simulink model "gtm_design"  (R2021b)
settings: Solver=VariableStepAuto  StartTime=0.0  StopTime=30  MinStep=0.0049  RelTol=1e-3
StopFcn:
  | MWSout=grabmws(bdroot);
  | MWSout.lastrun=datestr(now);
values from neighbouring files (symbols this model uses):
  g = 32.17405    [SingleDOF.m]    (also in layer1atm.m; mainSimple.m = 32.174; simio.m = [dx(Index.EOM(1:6)); delta(:)-f; -delta(:)-f ])
  GuidanceMode = 1    [mainSimple.m]    (also in setup.m)
  knots2fps = 1/fps2knots    (= 1.687800745)    [main.m]    (also in mainSimple.m = 1.68781)
  s = tf('s')    [SingleDOF.m]    (also in main.m; mainSimple.m; newmain.m)
undefined symbols (not defined in the file or in its folder): Aero, aftfuel, aftfuel_pos, AILL, AILLC, AILR, AILRC, alpha_deg, altitude_ft, Ax_g, Ay_g, Az_g, b, beta_deg, bias, BRAKEC, Cbar, cg_pos0, cg_shift_gear, DamageCase, DamageModels, DamageOnsetTime, Earth, ELLIB, ELLIBC, ELLOB, ELLOBC, ELRIB, ELRIBC, ELROB, ELROBC, engl_ang, engl_pos, engr_ang, engr_pos, FLAPLC, FLAPLIB, FLAPLOB, FLAPRC, FLAPRIB, FLAPROB, FuelUsed_Init, fwdfuel, fwdfuel_pos, GEAR, GEARC, Inertia0, Inertia_shift_gear, Ixx_model, Iyy_model, Izz_model, KTAS, LandingGear, LengON, LinearizeModeOn, m, MORPHLC, MORPHRC, NAV_altitude_m, NAV_latitude_deg ... (+51)
libraries: simulink_extras x39, simulink_need_slupdate x30, LPVBlockLibrary x9, aerolibconvert2 x7, simulink x3, aerolibtransform2 x3, UserContent_lib x2, uavalgslib x2, robotcorelib x1, uavutilslib x1
(part 7 of 7)

== system gtm_design/GTM_T2/Aero/Dynamic Derviatives/Rotary Blended UnDamaged Case/Forced Oscillation ==
  alpha : Inport
  pqr : Inport  Port=2
  Assignment to Lateral : Assignment  IndexMode=Zero-based  IndexOptions=Index vector (dialog)  Indices=[1 3 5]  OutputSizes=[1 1]
  Assignment to Lateral1 : Assignment  IndexMode=Zero-based  IndexOptions=Index vector (dialog)  Indices=[1 3 5]  OutputSizes=[1 1]
  Assignment to Longitudinal : Assignment  IndexMode=Zero-based  IndexOptions=Index vector (dialog)  Indices=[0 2 4]  OutputSizes=[1 1]
  Constant : Constant  Value=zeros(6,1)
  Constant1 : Constant  Value=[0:2]  OutDataTypeStr=uint32
  Constant2 : Constant  Value=[0:2]  OutDataTypeStr=uint32
  Constant3 : Constant  Value=[0:2]  OutDataTypeStr=uint32
  Constant4 : Constant  Value=zeros(6,1)
  Constant5 : Constant  Value=zeros(6,1)
  Demux : Demux  Outputs=3
  PreLookup Index Search : simulink_need_slupdate/PreLookup Index Search  bpData=Aero.dC3_q.alpha  searchMode=Binary Search  cacheBpFlag=on  outputFlag=off  IndexDataType=uint32  extrapMode=Linear Extrapolation  rangeErrorMode=None
      settings: SourceProductBaseCode=SL
  PreLookup Index Search1 : simulink_need_slupdate/PreLookup Index Search  bpData=Aero.dC3_r.rhat  searchMode=Binary Search  cacheBpFlag=on  outputFlag=off  IndexDataType=uint32  extrapMode=Linear Extrapolation  rangeErrorMode=None
      settings: SourceProductBaseCode=SL
  PreLookup Index Search2 : simulink_need_slupdate/PreLookup Index Search  bpData=Aero.dC3_p.phat  searchMode=Binary Search  cacheBpFlag=on  outputFlag=off  IndexDataType=uint32  extrapMode=Linear Extrapolation  rangeErrorMode=None
      settings: SourceProductBaseCode=SL
  PreLookup Index Search3 : simulink_need_slupdate/PreLookup Index Search  bpData=Aero.dC3_q.qhat  searchMode=Binary Search  cacheBpFlag=on  outputFlag=off  IndexDataType=uint32  extrapMode=Linear Extrapolation  rangeErrorMode=None
      settings: SourceProductBaseCode=SL
  PreLookup Index Search4 : simulink_need_slupdate/PreLookup Index Search  bpData=Aero.dC3_p.alpha  searchMode=Binary Search  cacheBpFlag=on  outputFlag=off  IndexDataType=uint32  extrapMode=Linear Extrapolation  rangeErrorMode=None
      settings: SourceProductBaseCode=SL
  PreLookup Index Search5 : simulink_need_slupdate/PreLookup Index Search  bpData=Aero.dC3_r.alpha  searchMode=Binary Search  cacheBpFlag=on  outputFlag=off  IndexDataType=uint32  extrapMode=Linear Extrapolation  rangeErrorMode=None
      settings: SourceProductBaseCode=SL
  pitch : simulink_need_slupdate/Interpolation (n-D) using PreLookup  numDimsPopupSelect=3  explicitNumDims=2  table=Aero.dC3_q.data  interpMethod=Linear  extrapMethod=Linear  rangeErrorMode=None  NumSelectionDims=1
      settings: SourceProductBaseCode=SL
  roll : simulink_need_slupdate/Interpolation (n-D) using PreLookup  numDimsPopupSelect=3  explicitNumDims=2  table=Aero.dC3_p.data  interpMethod=Linear  extrapMethod=Linear  rangeErrorMode=None  NumSelectionDims=1
      settings: SourceProductBaseCode=SL
  yaw : simulink_need_slupdate/Interpolation (n-D) using PreLookup  numDimsPopupSelect=3  explicitNumDims=2  table=Aero.dC3_r.data  interpMethod=Linear  extrapMethod=Linear  rangeErrorMode=None  NumSelectionDims=1
      settings: SourceProductBaseCode=SL
  dC6_p : Outport
  dC6_q : Outport  Port=2
  dC6_r : Outport  Port=3
  wires:
  alpha/1 -> PreLookup Index Search4/1, PreLookup Index Search5/1, PreLookup Index Search/1
  pqr/1 -> Demux/1
  Constant1/1 -> pitch/3
  Demux/2 -> PreLookup Index Search3/1
  Demux/1 -> PreLookup Index Search2/1
  Demux/3 -> PreLookup Index Search1/1
  Constant2/1 -> roll/3
  Constant3/1 -> yaw/3
  Constant/1 -> Assignment to Longitudinal/1
  pitch/1 -> Assignment to Longitudinal/2
  roll/1 -> Assignment to Lateral/2
  Constant4/1 -> Assignment to Lateral/1
  Constant5/1 -> Assignment to Lateral1/1
  yaw/1 -> Assignment to Lateral1/2
  PreLookup Index Search1/1 -> yaw/2
  PreLookup Index Search2/1 -> roll/2
  PreLookup Index Search3/1 -> pitch/2
  Assignment to Lateral/1 -> dC6_p/1
  Assignment to Lateral1/1 -> dC6_r/1
  Assignment to Longitudinal/1 -> dC6_q/1
  PreLookup Index Search/1 -> pitch/1
  PreLookup Index Search4/1 -> roll/1
  PreLookup Index Search5/1 -> yaw/1

== system gtm_design/GTM_T2/Aero/Dynamic Derviatives/Rotary Blended UnDamaged Case/Rotary Balance ==
  alpha : Inport
  beta : Inport  Port=2
  w : Inport  Port=3
  Constant1 : Constant  Value=[0:5]  OutDataTypeStr=uint32
  PreLookup Index Search : simulink_need_slupdate/PreLookup Index Search  bpData=Aero.dC6_w.alpha  searchMode=Binary Search  cacheBpFlag=on  outputFlag=off  IndexDataType=uint32  extrapMode=Linear Extrapolation  rangeErrorMode=None
      settings: SourceProductBaseCode=SL
  PreLookup Index Search1 : simulink_need_slupdate/PreLookup Index Search  bpData=Aero.dC6_w.beta  searchMode=Binary Search  cacheBpFlag=on  outputFlag=off  IndexDataType=uint32  extrapMode=Linear Extrapolation  rangeErrorMode=None
      settings: SourceProductBaseCode=SL
  PreLookup Index Search2 : simulink_need_slupdate/PreLookup Index Search  bpData=Aero.dC6_w.what  searchMode=Binary Search  cacheBpFlag=on  outputFlag=off  IndexDataType=uint32  extrapMode=Linear Extrapolation  rangeErrorMode=None
      settings: SourceProductBaseCode=SL
  TableLookup : simulink_need_slupdate/Interpolation (n-D) using PreLookup  numDimsPopupSelect=4  explicitNumDims=2  table=Aero.dC6_w.data  interpMethod=Linear  extrapMethod=Linear  rangeErrorMode=None  NumSelectionDims=1
      settings: SourceProductBaseCode=SL
  dC6 : Outport
  wires:
  PreLookup Index Search/1 -> TableLookup/1
  beta/1 -> PreLookup Index Search1/1
  alpha/1 -> PreLookup Index Search/1
  TableLookup/1 -> dC6/1
  Constant1/1 -> TableLookup/4
  w/1 -> PreLookup Index Search2/1
  PreLookup Index Search1/1 -> TableLookup/3
  PreLookup Index Search2/1 -> TableLookup/2

== system gtm_design/GTM_T2/Sensors/Air Data/First Order Filter/Enabled Subsystem ==
  In : Inport
  tau : Inport  Port=2
  Enable : EnablePort
  Divide : Product  Inputs=*/
  Integrator : Integrator  InitialConditionSource=external  UpperSaturationLimit=POS_hi  LowerSaturationLimit=POS_lo
  Sum : Sum  Inputs=-+|  InputSameDT=on  SaturateOnIntegerOverflow=on  OutDataTypeStr=Inherit: Same as first input
  Out : Outport
  wires:
  Sum/1 -> Divide/1  "Error"
  In/1 -> Sum/2, Integrator/2
  Integrator/1 -> Out/1, Sum/1  "Y"
  tau/1 -> Divide/2
  Divide/1 -> Integrator/1  "Ydot"

== system gtm_design/GTM_T2/TransportDelay/Transport Delay on Bus/BusDelay/TimeDelay with IC feedthrough ==
  I : Inport
  Clock : Clock
  Switch : Switch  Criteria=u2 > Threshold  Threshold=TimeDelay
  Transport Delay : TransportDelay  DelayTime=TimeDelay
      settings: AttributesFormatString=%<DelayTime>
  O : Outport
  wires:
  I/1 -> Transport Delay/1, Switch/3
  Clock/1 -> Switch/2
  Switch/1 -> O/1
  Transport Delay/1 -> Switch/1

== system gtm_design/GTM_T2/TransportDelay/Transport Delay on Bus/BusDelay1/TimeDelay with IC feedthrough ==
  I : Inport
  Clock : Clock
  Switch : Switch  Criteria=u2 > Threshold  Threshold=TimeDelay
  Transport Delay : TransportDelay  DelayTime=TimeDelay
      settings: AttributesFormatString=%<DelayTime>
  O : Outport
  wires:
  I/1 -> Transport Delay/1, Switch/3
  Clock/1 -> Switch/2
  Switch/1 -> O/1
  Transport Delay/1 -> Switch/1

== system gtm_design/GTM_T2/TransportDelay/Transport Delay on Bus/BusDelay2/TimeDelay with IC feedthrough ==
  I : Inport
  Clock : Clock
  Switch : Switch  Criteria=u2 > Threshold  Threshold=TimeDelay
  Transport Delay : TransportDelay  DelayTime=TimeDelay
      settings: AttributesFormatString=%<DelayTime>
  O : Outport
  wires:
  I/1 -> Transport Delay/1, Switch/3
  Clock/1 -> Switch/2
  Switch/1 -> O/1
  Transport Delay/1 -> Switch/1

== system gtm_design/GTM_T2/TransportDelay/Transport Delay on Bus/BusDelay3/TimeDelay with IC feedthrough ==
  I : Inport
  Clock : Clock
  Switch : Switch  Criteria=u2 > Threshold  Threshold=TimeDelay
  Transport Delay : TransportDelay  DelayTime=TimeDelay
      settings: AttributesFormatString=%<DelayTime>
  O : Outport
  wires:
  I/1 -> Transport Delay/1, Switch/3
  Clock/1 -> Switch/2
  Switch/1 -> O/1
  Transport Delay/1 -> Switch/1

== system gtm_design/GTM_T2/TransportDelay/Transport Delay on Bus/BusDelay4/TimeDelay with IC feedthrough ==
  I : Inport
  Clock : Clock
  Switch : Switch  Criteria=u2 > Threshold  Threshold=TimeDelay
  Transport Delay : TransportDelay  DelayTime=TimeDelay
      settings: AttributesFormatString=%<DelayTime>
  O : Outport
  wires:
  I/1 -> Transport Delay/1, Switch/3
  Clock/1 -> Switch/2
  Switch/1 -> O/1
  Transport Delay/1 -> Switch/1

== system gtm_design/Control/Controller/Control Algorithm/Longitudinal Controller/Altitude Controller/Altitude Controller ==
  alt_c_ft : Inport
  feedback : Inport  Port=2
  An_c_g : Step  Time=5  Before=0.9968  After=0.9  SampleTime=0
  An_c_g1 : Step  Time=10  After=0.0968  SampleTime=0
  Constant : Constant  Commented=on
  Constant1 : Constant  Value=0.9968
  Gain : Gain  Gain=-1
  Sum : Sum  Inputs=|++
  Terminator : Terminator
  Terminator1 : Terminator
  Az_c_g : Outport
  wires:
  alt_c_ft/1 -> Terminator/1
  feedback/1 -> Terminator1/1
  Gain/1 -> Az_c_g/1  "Az_c_g"
  An_c_g/1 -> Sum/1
  An_c_g1/1 -> Sum/2
  Sum/1 -> Gain/1

== system gtm_design/Control/Controller/Control Algorithm/Longitudinal Controller/Altitude Controller/Normal Acceleration Controller ==
  Az_c_g : Inport
  feedback : Inport  Port=2
  Demux2 : Demux  Outputs=[2 1]
  Full Output : Subsystem
  LPV Controller : LPVBlockLibrary/LPVBlock  sys=K_lon_lpv  plist={'rho1_sas_param';'rho2_alt_param';'rho3_mor_param'}  x0=0
      settings: SourceProductName=LPVTools Blocks
  Mux : Mux  Inputs=2
  Scheduling Parameter : Subsystem
  Scope : Scope
  Scope1 : Scope
  Scope2 : Scope
  Sum : Sum  Inputs=|+-
  Sum1 : Sum  Inputs=|+-
  Sum2 : Sum  Inputs=|++
  Sum3 : Sum  Inputs=|+-
  Trim Command : Subsystem
  Trim Input : Subsystem
  Trim Output : Subsystem
  dele_c_deg : Scope
  feedback_1 : InportShadow  Port=2
  knotstofps : Gain  Gain=g
  ELLC : Outport
  wires:
  feedback/1 -> Scheduling Parameter/1(feedback)
  Mux/1 -> LPV Controller/1
  [rho] -> Trim Input/1(rho)
  LPV Controller/1 -> Sum2/1  "du"
  Scheduling Parameter/1(rho) -> [rho]
  Sum3/1 -> Scope2/1, Mux/1  "dy"
  Sum1/1 -> Demux2/1  "dx"
  Trim Input/1(dele_trim_deg) -> Sum2/2
  Sum2/1 -> ELLC/1, dele_c_deg/1  "u"
  feedback_1/1 -> Full Output/1(feedback)
  [rho] -> Trim Output/1(rho)
  Trim Output/1(y_eq) -> Sum1/2  "y_eq"
  [rho] -> LPV Controller/2
  Full Output/1(y) -> Sum1/1  "y"
  Az_c_g/1 -> knotstofps/1
  knotstofps/1 -> Sum/1  "Az_c_fps"
  Trim Command/1(Az_trim_fps) -> Sum/2
  Sum/1 -> Scope/1, Sum3/1
  Demux2/2 -> Sum3/2, Scope1/1
  Demux2/1 -> Mux/2

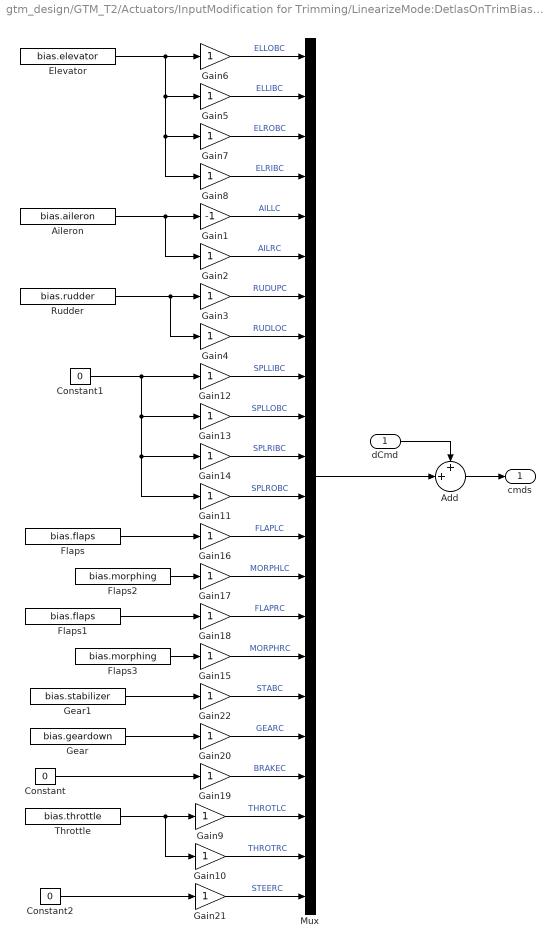
== system gtm_design/GTM_T2/Actuators/InputModification for Trimming/LinearizeMode:DetlasOnTrimBias/Surface Allocation For Linearizing/BiasSurfs ==
  dCmd : Inport
  Add : Sum  Inputs=++|
  Aileron : Constant  Value=bias.aileron
  Constant : Constant  Value=0
  Constant1 : Constant  Value=0
  Constant2 : Constant  Value=0
  Elevator : Constant  Value=bias.elevator
  Flaps : Constant  Value=bias.flaps
  Flaps1 : Constant  Value=bias.flaps
  Flaps2 : Constant  Value=bias.morphing
  Flaps3 : Constant  Value=bias.morphing
  Gain1 : Gain  Gain=-1  SaturateOnIntegerOverflow=on  OutDataTypeStr=Inherit: Same as input  ParamDataTypeStr=Inherit: Same as input
  Gain{2..22} (21 alike) : Gain  SaturateOnIntegerOverflow=on  OutDataTypeStr=Inherit: Same as input  ParamDataTypeStr=Inherit: Same as input
  Gear : Constant  Value=bias.geardown
  Gear1 : Constant  Value=bias.stabilizer
  Mux : Mux  Inputs=22
  Rudder : Constant  Value=bias.rudder
  Throttle : Constant  Value=bias.throttle
  cmds : Outport
  wires:
  Gain21/1 -> Mux/22  "STEERC"
  Constant2/1 -> Gain21/1
  Throttle/1 -> Gain10/1, Gain9/1
  Gain10/1 -> Mux/21  "THROTRC"
  Gain9/1 -> Mux/20  "THROTLC"
  Add/1 -> cmds/1
  dCmd/1 -> Add/1
  Mux/1 -> Add/2
  Gain22/1 -> Mux/17  "STABC"
  Gear1/1 -> Gain22/1
  Aileron/1 -> Gain2/1, Gain1/1
  Gain2/1 -> Mux/6  "AILRC"
  Gain1/1 -> Mux/5  "AILLC"
  Gain20/1 -> Mux/18  "GEARC"
  Constant/1 -> Gain19/1
  Gear/1 -> Gain20/1
  Gain19/1 -> Mux/19  "BRAKEC"
  Flaps/1 -> Gain16/1
  Rudder/1 -> Gain4/1, Gain3/1
  Elevator/1 -> Gain8/1, Gain7/1, Gain5/1, Gain6/1
  Gain4/1 -> Mux/8  "RUDLOC"
  Gain3/1 -> Mux/7  "RUDUPC"
  Gain8/1 -> Mux/4  "ELRIBC"
  Gain7/1 -> Mux/3  "ELROBC"
  Gain6/1 -> Mux/1  "ELLOBC"
  Gain5/1 -> Mux/2  "ELLIBC"
  Gain15/1 -> Mux/16  "MORPHRC"
  Gain18/1 -> Mux/15  "FLAPRC"
  Gain17/1 -> Mux/14  "MORPHLC"
  Gain16/1 -> Mux/13  "FLAPLC"
  Gain11/1 -> Mux/12  "SPLROBC"
  Gain14/1 -> Mux/11  "SPLRIBC"
  Gain13/1 -> Mux/10  "SPLLOBC"
  Gain12/1 -> Mux/9  "SPLLIBC"
  Constant1/1 -> Gain13/1, Gain11/1, Gain14/1, Gain12/1
  Flaps2/1 -> Gain17/1
  Flaps1/1 -> Gain18/1
  Flaps3/1 -> Gain15/1

== system gtm_design/GTM_T2/Actuators/InputModification for Trimming/TrimMode: DriveFromTopLevel/MapPitchSurf/UseElevatorToTrim ==
  In : Inport
  Action Port : ActionPort  ActionPortLabel=default:
  Constant1 : Constant  Value=bias.stabilizer
  Gain : Gain  Gain=[1;1;1;1]
  Mux : Mux  Inputs=[4 1]
  Out : Outport  InitialOutput=[0;0;0;0;bias.stabilizer]
  wires:
  Mux/1 -> Out/1
  Gain/1 -> Mux/1
  Constant1/1 -> Mux/2
  In/1 -> Gain/1

== system gtm_design/GTM_T2/Actuators/InputModification for Trimming/TrimMode: DriveFromTopLevel/MapPitchSurf/UseStabToTrim ==
  In : Inport
  Action Port : ActionPort  ActionPortLabel=case [ 1 ]:
  Constant1 : Constant  Value=bias.elevator
  Gain2 : Gain  Gain=[1;1;1;1]
  Mux : Mux  Inputs=[4 1]
  Out1 : Outport  InitialOutput=[bias.elevator*[1;1;1;1];0]
  wires:
  Mux/1 -> Out1/1
  Gain2/1 -> Mux/1
  In/1 -> Mux/2
  Constant1/1 -> Gain2/1

== system gtm_design/Control/Controller/Control Algorithm/Longitudinal Controller/Altitude Controller/Normal Acceleration Controller/Full Output ==
  feedback : Inport
  Az_g : Scope
  Bus Selector : BusSelector  OutputSignals=AirData.alpha_deg,MAG3.q_deg,MAG3.Az_g
  Degrees to Radians : simulink_extras/Transformations/Degrees to Radians
  Degrees to Radians1 : simulink_extras/Transformations/Degrees to Radians
  Mux : Mux  Inputs=3
  alpha_deg : Scope
  knotstofps : Gain  Gain=g
  q_deg : Scope
  y : Outport
  wires:
  feedback/1 -> Bus Selector/1
  Bus Selector/1 -> alpha_deg/1, Degrees to Radians/1  "<alpha_deg>"
  Bus Selector/2 -> q_deg/1, Degrees to Radians1/1  "<q_deg>"
  Bus Selector/3 -> knotstofps/1, Az_g/1  "<Az_g>"
  Degrees to Radians1/1 -> Mux/2  "q_rad"
  Degrees to Radians/1 -> Mux/1  "alp_rad"
  knotstofps/1 -> Mux/3  "Az_fps"
  Mux/1 -> y/1

== system gtm_design/Control/Controller/Control Algorithm/Longitudinal Controller/Altitude Controller/Normal Acceleration Controller/Scheduling Parameter ==
  feedback : Inport
  Add : Sum
  Bus Selector1 : BusSelector  OutputSignals=AirData.KTAS,MIDG.NAV_altitude_m,SurfacePos.FLAPLOB,SurfacePos.FLAPROB  OutputAsBus=on
  Bus to Vector : BusToVector
  Demux : Demux
  Gain : Gain  Gain=0.5
  Length Conversion : aerolibconvert2/Length Conversion  IU=m  OU=ft
  MATLAB Function : MATLAB Function  TreatAsAtomicUnit=on
  Mux : Mux  Inputs=3
  rho : Outport
  wires:
  feedback/1 -> Bus Selector1/1
  Bus Selector1/1 -> Bus to Vector/1
  Demux/3 -> Add/1
  Demux/1 -> MATLAB Function/1(tas)
  Demux/4 -> Add/2
  MATLAB Function/1(sas) -> Mux/1  "sas"
  Add/1 -> Gain/1
  Gain/1 -> Mux/3  "mor"
  Demux/2 -> Length Conversion/1  "alt"
  Bus to Vector/1 -> Demux/1
  Mux/1 -> rho/1
  Length Conversion/1 -> MATLAB Function/2(h), Mux/2

== system gtm_design/Control/Controller/Control Algorithm/Longitudinal Controller/Altitude Controller/Normal Acceleration Controller/Trim Command ==
  Constant : Constant  Value=-1
  knotstofps : Gain  Gain=g
  Az_trim_fps : Outport
  wires:
  knotstofps/1 -> Az_trim_fps/1  "Az_c_fps"
  Constant/1 -> knotstofps/1

== system gtm_design/Control/Controller/Control Algorithm/Longitudinal Controller/Altitude Controller/Normal Acceleration Controller/Trim Input ==
  rho : Inport
  Constant3 : Constant
  Scope1 : Scope
  dele_trim : LPVBlockLibrary/LPVBlock  sys=sch_elevator_trim  plist={'rho1_sas_param';'rho2_alt_param';'rho3_mor_param'}  x0=0
      settings: SourceProductName=LPVTools Blocks
  dele_trim_deg : Outport
  wires:
  Constant3/1 -> dele_trim/1
  dele_trim/1 -> dele_trim_deg/1, Scope1/1  "dele_trim_deg"
  rho/1 -> dele_trim/2

== system gtm_design/Control/Controller/Control Algorithm/Longitudinal Controller/Altitude Controller/Normal Acceleration Controller/Trim Output ==
  rho : Inport
  Constant1 : Constant  Value=0
  Constant2 : Constant
  Constant3 : Constant  Value=-1
  Degrees to Radians : simulink_extras/Transformations/Degrees to Radians
  LPVBlock : LPVBlockLibrary/LPVBlock  sys=sch_alp_trim  plist={'rho1_sas_param';'rho2_alt_param';'rho3_mor_param'}  x0=0
      settings: SourceProductName=LPVTools Blocks
  Mux : Mux  Inputs=3
  Scope : Scope
  knotstofps : Gain  Gain=g
  y_eq : Outport
  wires:
  Degrees to Radians/1 -> Mux/1  "alp_trim_rad"
  Constant2/1 -> LPVBlock/1
  LPVBlock/1 -> Scope/1, Degrees to Radians/1  "alp_trim_deg"
  Constant1/1 -> Mux/2  "q_trim_rad"
  knotstofps/1 -> Mux/3  "Az_trim_fps"
  rho/1 -> LPVBlock/2
  Constant3/1 -> knotstofps/1  "Az_trim_g"
  Mux/1 -> y_eq/1

== matlab function gtm_design/GTM_T2/EOM/Aircraft 6DOF/Form Inertia Matrix ==
  data: Ixx input double size=1; I output size=[3 3]; Iyy input size=1; Izz input size=1; Ixz input size=1; Iyz input size=1; Ixy input size=1; InvI output size=[3 3]
function [I,InvI] = Inertia(Ixx,Iyy,Izz,Ixz,Iyz,Ixy)
% This block supports an embeddable subset of the MATLAB language.
% See the help menu for details. 

I=[ Ixx, -Ixy, -Ixz;
   -Ixy,  Iyy, -Iyz;
   -Ixz, -Iyz,   Izz ];

det = Ixx*Iyy*Izz-Ixx*Iyz^2-Ixy^2*Izz-2*Ixy*Ixz*Iyz-Ixz^2*Iyy;

adjoint=[...
Iyy*Izz-Iyz^2,    Ixy*Izz+Ixz*Iyz, Ixy*Iyz+Ixz*Iyy;...
Ixy*Izz+Ixz*Iyz,   Ixx*Izz-Ixz^2,  Ixx*Iyz+Ixy*Ixz;...
Ixy*Iyz+Ixz*Iyy,  Ixx*Iyz+Ixy*Ixz,   Ixx*Iyy-Ixy^2     ];

InvI=adjoint/det;

== matlab function gtm_design/GTM_T2/Engines/Engine Alignment ==
  data: T output; Tl input; hl input; Tr input; hr input; TL output; engl_ang parameter; engr_ang parameter; TR output; H output
function [T,TL,TR,H] = eng_angles(Tl,hl,Tr,hr,engl_ang,engr_ang)
% This block supports an embeddable subset of the MATLAB language.
% See the help menu for details. 

% Using the engine alignment angles (set in AC_params_T2.m), compute the 
% off-axis thrust and angular momentum terms.

TL = Tl*[cosd(engl_ang(2))*cosd(engl_ang(3));...
         sind(engl_ang(3));...
         -sind(engl_ang(2))*cosd(engl_ang(3))];
TR = Tr*[cosd(engr_ang(2))*cosd(engr_ang(3));...
         sind(engr_ang(3));...
         -sind(engr_ang(2))*cosd(engr_ang(3))];  
T = TL+TR;

H = hl*[cosd(engl_ang(2))*cosd(engl_ang(3));...
         sind(engl_ang(3));...
         -sind(engl_ang(2))*cosd(engl_ang(3))] + ...
         hr*[cosd(engr_ang(2))*cosd(engr_ang(3));...
         sind(engr_ang(3));...
         -sind(engr_ang(2))*cosd(engr_ang(3))];

== matlab function gtm_design/GTM_T2/Engines/Left_Engine Jetcat P70/Simple Ram Drag Model ==
  data: ram_drag output; qbar input; S input; ram_drag_coef parameter
function ram_drag =   ram_drag(qbar,S,ram_drag_coef)
% This block supports the Embedded MATLAB subset.
% See the help menu for details. 

ram_drag = ram_drag_coef.*qbar.*S;
return

== matlab function gtm_design/GTM_T2/Engines/Right_Engine Jetcat P70/Simple Ram Drag Model ==
  data: ram_drag output; qbar input; S input; ram_drag_coef parameter
function ram_drag =   ram_drag(qbar,S,ram_drag_coef)
% This block supports the Embedded MATLAB subset.
% See the help menu for details. 

ram_drag = ram_drag_coef.*qbar.*S;
return

== matlab function gtm_design/Control/Controller/Control Algorithm/Longitudinal Controller (Gamma)/Scheduling Parameter/MATLAB Function ==
  data: tas input; sas output; h input
function sas = fcn(tas, h)
sas = 100-30000/(30000-h)*(100-tas);

== matlab function gtm_design/GTM_T2/A/C parameters/Inertia/Mass/CG Shift/FuelBurnEffects/Polyval1/Embedded MATLAB Function ==
  data: u input; y output; p parameter
function y = fcn(u,p)
% This block supports the Embedded MATLAB subset.
% See the help menu for details. 


y = sum(p.*u.^(length(p)-1:-1:0));

== matlab function gtm_design/Control/Controller/Control Algorithm/Longitudinal Controller (Gamma)/Trim Command/MATLAB Function ==
  data: sas input; tas output; h input
function tas = fcn(sas,h)

tas = 100-(30000-h)/30000*(100-sas);

== matlab function gtm_design/Control/Controller/Control Algorithm/Lateral-Directional Controller/Scheduling Parameter/MATLAB Function ==
  data: tas input; sas output; h input
function sas = fcn(tas, h)
sas = 100-30000/(30000-h)*(100-tas);

== matlab function gtm_design/GTM_T2/A//C parameters/Inertia//Mass//CG Shift/MorphingEffects/MorphingEffectsInertia ==
  data: fuel_used input; y output; aftfuel parameter; fwdfuel parameter; aftfuel_pos parameter; fwdfuel_pos parameter; w0 parameter; cg_pos0 parameter
function y = fcn(fuel_used,aftfuel,fwdfuel,aftfuel_pos,fwdfuel_pos,w0,cg_pos0)
% This block supports an embeddable subset of the MATLAB language.
% See the help menu for details. 

y = w0.*cg_pos0 - min(aftfuel,fuel_used).*aftfuel_pos - max(0,fuel_used-fwdfuel).*fwdfuel_pos;

== matlab function gtm_design/GTM_T2/A//C parameters/Inertia//Mass//CG Shift/MorphingEffects1/MorphingEffectsCG ==
  data: fuel_used input; y output; aftfuel parameter; fwdfuel parameter; aftfuel_pos parameter; fwdfuel_pos parameter; w0 parameter; cg_pos0 parameter
function y = fcn(fuel_used,aftfuel,fwdfuel,aftfuel_pos,fwdfuel_pos,w0,cg_pos0)
% This block supports an embeddable subset of the MATLAB language.
% See the help menu for details. 

y = w0.*cg_pos0 - min(aftfuel,fuel_used).*aftfuel_pos - max(0,fuel_used-fwdfuel).*fwdfuel_pos;

== matlab function gtm_design/Control/Controller/Control Algorithm/Longitudinal Controller (Gamma)/Trim State/MATLAB Function ==
  data: sas input; tas output; h input
function tas = fcn(sas,h)

tas = 100-(30000-h)/30000*(100-sas);

== matlab function gtm_design/Guidance/Orbit Following/Heading Control ==
  data: FlightState input Bus: FixedWingStateBus; UHeading input; RollAngle output size=[1 1]; e input Bus: FixedWingEnvironmentBus
function RollAngle = fcn(FlightState, UHeading, e)

PHeadingAngle = 0.39;

Va = FlightState.AirSpeed;
HeadingAngle = FlightState.HeadingAngle;
FlightPathAngle = FlightState.FlightPathAngle;

YawAngle = HeadingAngle - asin((1/Va)*[e.WindNorth, e.WindEast]*[-sin(HeadingAngle); cos(HeadingAngle)]);
b = [cos(HeadingAngle)*cos(FlightPathAngle), sin(HeadingAngle)*cos(FlightPathAngle), -sin(FlightPathAngle)]*[e.WindNorth; e.WindEast; e.WindDown];
c = [e.WindNorth, e.WindEast, e.WindDown]*[e.WindNorth; e.WindEast; e.WindDown]- Va^2;
Vg = -b+sqrt(b^2-c);

RollAngle = atan2(PHeadingAngle*angdiff(HeadingAngle,UHeading)*Vg,e.Gravity*cos(HeadingAngle-YawAngle));

== matlab function gtm_design/Guidance/Waypoint Following/Heading Control ==
  data: FlightState input Bus: FixedWingStateBus; UHeading input; RollAngle output size=[1 1]; e input Bus: FixedWingEnvironmentBus
function RollAngle = fcn(FlightState, UHeading, e)

PHeadingAngle = 0.39;

Va = FlightState.AirSpeed;
HeadingAngle = FlightState.HeadingAngle;
FlightPathAngle = FlightState.FlightPathAngle;

YawAngle = HeadingAngle - asin((1/Va)*[e.WindNorth, e.WindEast]*[-sin(HeadingAngle); cos(HeadingAngle)]);
b = [cos(HeadingAngle)*cos(FlightPathAngle), sin(HeadingAngle)*cos(FlightPathAngle), -sin(FlightPathAngle)]*[e.WindNorth; e.WindEast; e.WindDown];
c = [e.WindNorth, e.WindEast, e.WindDown]*[e.WindNorth; e.WindEast; e.WindDown]- Va^2;
Vg = -b+sqrt(b^2-c);

RollAngle = atan2(PHeadingAngle*angdiff(HeadingAngle,UHeading)*Vg,e.Gravity*cos(HeadingAngle-YawAngle));

== matlab function gtm_design/Control/Controller/Control Algorithm/Longitudinal Controller/Altitude Controller/Normal Acceleration Controller/Scheduling Parameter/MATLAB Function ==
  data: tas input; sas output; h input
function sas = fcn(tas, h)
sas = 100-30000/(30000-h)*(100-tas);

== matlab function gtm_design/GTM_T2/A/C parameters/Inertia/Mass/CG Shift/fuel cg shift, cg_pos0 ==
  data: fuel_used input; y output; aftfuel parameter; fwdfuel parameter; aftfuel_pos parameter; fwdfuel_pos parameter; w0 parameter; cg_pos0 parameter
function y = fcn(fuel_used,aftfuel,fwdfuel,aftfuel_pos,fwdfuel_pos,w0,cg_pos0)
% This block supports an embeddable subset of the MATLAB language.
% See the help menu for details. 

y = w0.*cg_pos0 - min(aftfuel,fuel_used).*aftfuel_pos - max(0,fuel_used-fwdfuel).*fwdfuel_pos;

== matlab function gtm_design/GTM_T2/A/C parameters/Inertia/Mass/CG Shift/FuelBurnEffects/Polyval2/Embedded MATLAB Function ==
  data: u input; y output; p parameter
function y = fcn(u,p)
% This block supports the Embedded MATLAB subset.
% See the help menu for details. 


y = sum(p.*u.^(length(p)-1:-1:0));

== matlab function gtm_design/GTM_T2/Aero/Control Surfaces/Implement Damage Models/Implement Damage Models ==
  data: SurfVec input; DamageCase input; dC6 output; SurfGain parameter
function dC6 = fcn(SurfVec,DamageCase,SurfGain)
% This block supports an embeddable subset of the MATLAB language.
% See the help menu for details. 
damagecase = cast(round(DamageCase),'uint32');
Nsurfs=18;
if (damagecase==0),
    dC6=ones(1,Nsurfs)*(reshape(SurfVec,6,Nsurfs)');
else
  gain=squeeze(SurfGain(damagecase,:,:));
  dC6=ones(1,Nsurfs)*( transpose(reshape(SurfVec,6,Nsurfs)).*gain);
end

== matlab function gtm_design/GTM_T2/Aero/Dynamic Derviatives/Rotary Blended UnDamaged Case/Blending Function ==
  data: alpha input; omega output; beta input; tas input; pqr input; pqr_osc output; B input; Cbar input
function[omega,pqr_osc]= hykal(alpha,beta,tas,pqr,B,Cbar)
% Hybrid Kalviste blending method for use in embedded block in Simulink.
%
% Austin Murch
% Austin.M.Murch@nasa.gov

% Dimension vector outputs.
pqr_osc=zeros(3,1);
 

% Constants
dtr=pi/180;
knots2ft=1.689;

% Setup variables
pb=pqr(1);
qb=pqr(2);
rb=pqr(3);

alpha = alpha*dtr;
beta = beta*dtr;
omega = 0;

%----Hybrid Kalviste Method----%
whichcase = 0;

%Test for case 1: p_osc = 0
if cos(alpha)*cos(beta) == 0
elseif pb == 0
else
    omega = pb/(cos(alpha)*cos(beta));
    r_osc = rb - omega*sin(alpha)*cos(beta);
    if abs(r_osc) > abs(rb)
    elseif r_osc*rb < 0
    else
        whichcase = 1;
    end
end

%Test for case 2: r_osc = 0
if sin(alpha)*cos(beta) == 0
elseif rb == 0
else
    omega = rb/(sin(alpha)*cos(beta));
    p_osc = pb - omega*cos(alpha)*cos(beta);
    if abs(p_osc) > abs(pb)
    elseif p_osc*pb < 0
    else
        whichcase = 2;
    end
end

%Test for case 3: Omega = 0
if whichcase == 0
    whichcase = 3;
end

 

switch whichcase
    case 1
        omega = pb/(cos(alpha)*cos(beta));
        pqr_osc(1) = 0;        
        pqr_osc(2) = qb - omega*sin(beta);        
        pqr_osc(3) = rb - omega*sin(alpha)*cos(beta);

    case 2
        omega = rb/(sin(alpha)*cos(beta));
        pqr_osc(1) = pb - omega*cos(alpha)*cos(beta);
        pqr_osc(2) = qb - omega*sin(beta);
        pqr_osc(3) = 0;

    case 3
        pqr_osc(1) = pb;
        pqr_osc(2) = qb;
        pqr_osc(3) = rb;
        omega = 0;
end

%-----------------------------------------------% End Hybrid Kalviste

% Scale values for table lookup
b2vt=B/(2*tas*knots2ft);
c2vt=Cbar/(2*tas*knots2ft);
omega=omega*b2vt;
pqr_osc=pqr_osc.*[b2vt;c2vt;b2vt];

== matlab function gtm_design/GTM_T2/A/C parameters/Inertia/Mass/CG Shift/FuelBurnEffects/Polyval/Embedded MATLAB Function ==
  data: u input; y output; p parameter
function y = fcn(u,p)
% This block supports the Embedded MATLAB subset.
% See the help menu for details. 


y = sum(p.*u.^(length(p)-1:-1:0));

== matlab function gtm_design/GTM_T2/AuxiliaryVariables/Atmos76/atmos76 ==
  data: z input; y output; dt input
function y = layer1atm(z,dt)
% Author: Kevin Cunningham          April 20, 1992    
% Modified: Dave Cox                Aug, 14, 2008

y=zeros(6,1);

%dt=0;  % Standard Temp forced.

%    --- constants from 1976 std. atmosphere
r     = 1716.55915670803;
gamma = 1.4;
g     = 32.17405;
re    = 20855531.5;
tsl   = 288.15 * 1.8;
psl   = 2116.22;
hsl   = 0.;
sldens = 0.0023769;                 % atmospheric density at sea level
slpr   = 2116.220;                  % sea level pressure, psf

%---------------------------------------------------------------------
%    conversion from metric lapse rate to english lapse rate
%    meters/0.3048 = ft
%    Kelvin * 1.8 = Rankine
rm2ft = 1000.0/0.3048;
conlapse = 1.8/rm2ft;

%  ---- convert geometric alt. to geopotential alt.
h     = (re*z)/(re+z);
 
%  ---- ensure we are in layer one (based on geopotential alt)
if (h > 11*rm2ft) % 11 km
  %fprintf(1,'Error, atmosphere model out of range %f, Limiting...\n',h);
  h=11*rm2ft;
end
if (h<0)
  %fprintf(1,'Error, atmosphere model out of range %f, Limiting...\n',h);
  h=0;
end

a1     = -6.5*conlapse;
t1     = tsl + a1*(h-hsl);
del1   = (t1/tsl)^(-g/r/a1);
p1     = del1 * psl;

%   ---- apply temperature increment from standard day*/
t1     = t1 + dt;

%   ---- calculate density from eqn. of state w/ corrected temp.*/
rho1   = p1 / (r * t1);
 
%   ---- calculate speed of sound w/ corrected temp.*/
c1     = sqrt(gamma * (r * t1));
 

% Calculate outputs
y(1) = rho1;
y(2) = p1;
y(3) = t1 / 1.8; % output temperature  in Kelvin
y(4) = c1;
y(5) = y(2) / slpr;         % pressure ratio
y(6) = sqrt(y(1)/sldens);   % SQUARE ROOT OF DENSITY RATIO

== matlab function gtm_design/GTM_T2/AuxiliaryVariables/Embedded MATLAB Function ==
  data: omega input; euler input; v input; n_body output; v_dot input
function n_body = accels(omega,euler,v,v_dot)
% Compute body-axis accelerometer measurements.  
% Inputs:
%       omega: body-axis angular rates, [p q r], in rad/sec
%       euler: Euler angles, [phi theta psi], in rad
%           v: body-axis velocities, [u v w], ft/sec
%       v_dot: body-axis accelerations, [udot vdot wdot], ft/sec^2
%
%
% Author: Austin Murch (Austin.M.Murch@nasa.gov)
% Created: 2/19/2008

g0    = 32.174;
phi   = euler(1);
theta = euler(2);

n_body = (v_dot + cross(omega,v))/g0 - [-sin(theta); cos(theta)*sin(phi); cos(theta)*cos(phi)];

== matlab function gtm_design/GTM_T2/EOM/Aircraft 6DOF/EulerDot ==
  data: pqr input size=3; deuler output size=3; euler input size=3
function deuler = e2de(pqr,euler)
% This block supports an embeddable subset of the MATLAB language.
% See the help menu for details. 

P=pqr(1);
Q=pqr(2);
R=pqr(3);

phi=euler(1);
theta=euler(2);
psi=euler(3);

c_phi=cos(phi);
s_phi=sin(phi);
c_theta=cos(theta);
s_theta=sin(theta);

phi_dot   = P + (1/c_theta)*(s_phi*s_theta*Q + c_phi*s_theta*R);
theta_dot = c_phi*Q - s_phi*R;
psi_dot   = (1/c_theta)*(s_phi*Q + c_phi*R);

deuler=[phi_dot; theta_dot; psi_dot];
